simulink model "FSC_integral_KF"  (R2024b)
settings: Solver=FixedStepAuto  StartTime=0.0  StopTime=inf  FixedStep=0.001  RelTol=1e-3  EnableMultiTasking=on
undefined symbols (not defined in the file or in its folder): DiscIntNeverNeededParam, Discrete, Time
libraries: px4Sensorslib x5, px4Peripheralslib x1, ctrlSharedLib x1, cstblocks x1
settings Model: SimulationMode=external  ExtModeTrigDuration=10  Creator=ArriGE66  LastModifiedBy=xippa
settings SolverCC: PositivePriorityOrder=on
settings OptimizationCC: EnhancedBackFolding=on  PassReuseOutputArgsAs=Individual arguments  ZeroExternalMemoryAtStartup=off  ZeroInternalMemoryAtStartup=off  MaxStackSize=64  OptimizeBlockOrder=speed  DifferentSizesBufferReuse=on  OptimizationCustomize=off  EfficientTunableParamExpr=on
settings DebuggingCC: ParameterTunabilityLossMsg=error
settings HardwareCC: ProdBitPerPointer=32  ProdBitPerSizeT=32  ProdBitPerPtrDiffT=32  ProdLargestAtomicInteger=Long  ProdLargestAtomicFloat=Double  ProdWordSize=32  ProdLongLongMode=on  ProdHWDeviceType=ARM Compatible->ARM Cortex
settings SFSimCC: MATLABDynamicMemAlloc=off  SimTargetLang=C++
settings RTWCC: Description=Embedded Coder  SystemTargetFile=ert.tlc  HardwareBoard=PX4 Cube Orange  TemplateMakefile=ert_default_tmf  Toolchain=GNU Tools for PX4 Autopilots  TargetLang=C++  GPUComputeCapability=3.5
settings CodeAppCC: ForceParamTrailComments=on  IgnoreCustomStorageClasses=off  OperatorAnnotations=on  SimulinkDataObjDesc=on  SFDataObjDesc=on  InsertBlockDesc=on
settings ERTTargetCC: SupportVariableSizeSignals=on  ExtMode=on  ExtModeTransport=3  ExtModeStaticAlloc=on  ExtModeStaticAllocSize=1024  ExtModeMexFile=ext_xcp  ExtModeMexArgs=1 COM10 3000000  ExtModeIntrfLevel=Level2 - Open  InlinedParameterPlacement=Hierarchical  DynamicArrayContainerType=coder::array

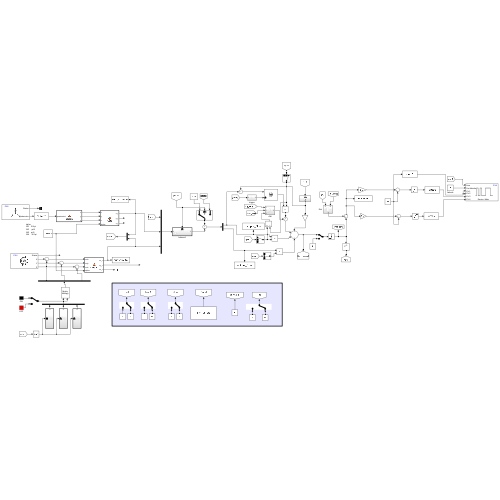
[thumbnail: Simulink's stored preview of the top-level diagram]
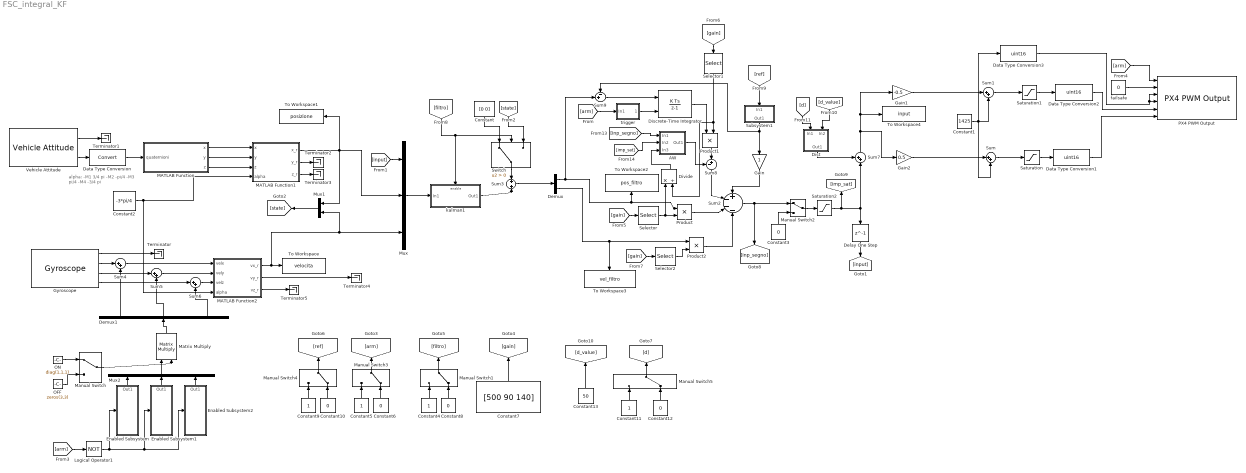
== system FSC_integral_KF ==
  note: alpha:
      | -M1    3/4 pi
      | -M2    -pi/4
      | -M3    pi/4
      | -M4    -3/4 pi
  " AW" : Subsystem
  Constant : Constant  Value=[0 0]
  Constant1 : Constant  Value=1425  SampleTime=0.01
  Constant{3,6,8,10,12} (5 alike) : Constant  Value=0
  Constant{4..5,9,11} (4 alike) : Constant
  Constant13 : Constant  Value=50
  Constant2 : Constant  Value=-3*pi/4  SampleTime=0.01
  Constant7 : Constant  Value=[500 90 140]
  Data Type Conversion : DataTypeConversion  SaturateOnIntegerOverflow=off  RndMeth=Floor
  Data Type Conversion1 : DataTypeConversion  OutDataTypeStr=uint16  SaturateOnIntegerOverflow=off  RndMeth=Floor
  Data Type Conversion2 : DataTypeConversion  OutDataTypeStr=uint16  SaturateOnIntegerOverflow=off  RndMeth=Floor
  Data Type Conversion3 : DataTypeConversion  OutDataTypeStr=uint16  SaturateOnIntegerOverflow=off  RndMeth=Floor
  Delay One Step : Delay  DelayLength=1
  Demux : Demux  Outputs=2
  Demux1 : Demux  Outputs=3
  Discrete-Time Integrator : DiscreteIntegrator  ExternalReset=level  SampleTime=-1  ICPrevOutput=DiscIntNeverNeededParam  ICPrevScaledInput=DiscIntNeverNeededParam
  Dist : Subsystem
  Divide : Product  Inputs=*/
  Enabled Subsystem : Subsystem  TreatAsAtomicUnit=on
  Enabled Subsystem1 : Subsystem  TreatAsAtomicUnit=on
  Enabled Subsystem2 : Subsystem  TreatAsAtomicUnit=on
  Gain : Gain
  Gain1 : Gain  Gain=-0.5
  Gain2 : Gain  Gain=0.5
  Gyroscope : px4Sensorslib/Gyroscope  uorbTimeStamp=off  BlockingMode=off  BlockTimeout=1e-3  sampleTime=0.01
  Logical Operator1 : Logic  Operator=NOT  AllPortsSameDT=off  OutDataTypeStr=boolean
  MATLAB Function : MATLAB Function  TreatAsAtomicUnit=on
  MATLAB Function1 : MATLAB Function  TreatAsAtomicUnit=on
  MATLAB Function2 : MATLAB Function  TreatAsAtomicUnit=on
  Manual Switch : ManualSwitch
  Manual Switch{1,3..5} (4 alike) : ManualSwitch  CurrentSetting=0
  Manual Switch2 : ManualSwitch
  Matrix Multiply : Product  Multiplication=Matrix(*)
  Mux : Mux  Inputs=3
  Mux1 : Mux  Inputs=2
  Mux2 : Mux  Inputs=3
  OFF : Constant  Value=zeros(3,3)
  ON : Constant  Value=diag(1,1,1)
  PX4 PWM Output : px4Peripheralslib/PX4 PWM Output  pwmDevice=Main  pwmChannel1_=on  pwmChannel2_=on  pwmChannel3_=on  pwmChannel4_=on  pwmChannel5_=off  pwmChannel6_=off  pwmChannel7_=off  pwmChannel8_=off
  Product : Product
  Product1 : Product
  Product2 : Product
  Saturation : Saturate  UpperLimit=1750  LowerLimit=1050
  Saturation1 : Saturate  UpperLimit=1750  LowerLimit=1050
  Saturation2 : Saturate  UpperLimit=600  LowerLimit=-600
  Selector : Selector  InputPortWidth=3  IndexOptions=Index vector (dialog)  Indices=1  OutputSizes=1
  Selector1 : Selector  InputPortWidth=3  IndexOptions=Index vector (dialog)  Indices=3  OutputSizes=1
  Selector2 : Selector  InputPortWidth=3  IndexOptions=Index vector (dialog)  Indices=2  OutputSizes=1
  Subsystem1 : Subsystem
  Sum{,1,4..6} (5 alike) : Sum  Inputs=|++
  Sum2 : Sum  Inputs=+---
  Sum3 : Sum
  Sum7 : Sum  Inputs=++|
  Sum8 : Sum  Inputs=-+|
  Sum9 : Sum  Inputs=-+|
  Switch : Switch  Criteria=u2 > Threshold  SaturateOnIntegerOverflow=off  InputSameDT=off
  Terminator{,1..5} (6 alike) : Terminator
  To Workspace : ToWorkspace  VariableName=velocita  SaveFormat=Timeseries  SampleTime=-1
  To Workspace1 : ToWorkspace  VariableName=posizione  SaveFormat=Timeseries  SampleTime=-1
  To Workspace2 : ToWorkspace  VariableName=pos_filtro  SaveFormat=Timeseries  SampleTime=-1
  To Workspace3 : ToWorkspace  VariableName=vel_filtro  SaveFormat=Timeseries  SampleTime=-1
  To Workspace4 : ToWorkspace  VariableName=input  SaveFormat=Timeseries  SampleTime=-1
  Vehicle Attitude : px4Sensorslib/Vehicle Attitude  rollRate=off  pitchRate=off  yawRate=off  quaternion=on  uorbTimeStamp=off  BlockingMode=off  BlockTimeout=0.001  sampleTime=0.01
  failsafe : Constant  Value=0  OutDataTypeStr=boolean  SampleTime=0.01
  kalman1 : Subsystem  TreatAsAtomicUnit=on
  trigger : Subsystem
  wires:
  Gain1/1 -> Sum1/1
  Data Type Conversion2/1 -> PX4 PWM Output/5
  Sum/1 -> Saturation/1
  Gain2/1 -> Sum/1
  MATLAB Function/2(y) -> MATLAB Function1/2(y)
  MATLAB Function/1(x) -> MATLAB Function1/1(x)
  MATLAB Function/3(z) -> MATLAB Function1/3(z)
  Constant1/1 -> Data Type Conversion3/1, Sum1/2, Sum/2
  Data Type Conversion1/1 -> PX4 PWM Output/6
  failsafe/1 -> PX4 PWM Output/2
  Sum1/1 -> Saturation1/1
  Vehicle Attitude/2 -> Data Type Conversion/1
  Data Type Conversion3/1 -> PX4 PWM Output/3, PX4 PWM Output/4
  MATLAB Function2/1(vx_r) -> To Workspace/1, Mux/3, Mux1/2
  Vehicle Attitude/1 -> Terminator1/1
  Saturation/1 -> Data Type Conversion1/1
  Saturation1/1 -> Data Type Conversion2/1
  MATLAB Function1/3(z_r) -> Terminator3/1
  MATLAB Function1/2(y_r) -> Terminator2/1
  MATLAB Function2/3(vz_r) -> Terminator5/1
  MATLAB Function2/2(vy_r) -> Terminator4/1
  Product/1 -> Sum2/3
  MATLAB Function1/1(x_r) -> To Workspace1/1, Mux/2, Mux1/1
  Mux/1 -> kalman1/1(In1)
  kalman1/1(Out1) -> Sum3/2
  Sum3/1 -> Demux/1
  Demux/2 -> Product2/1, To Workspace3/1
  Sum6/1 -> MATLAB Function2/3(velz)
  Gyroscope/1 -> Terminator/1
  Gyroscope/4 -> Sum6/1
  Sum4/1 -> MATLAB Function2/1(velx)
  Sum5/1 -> MATLAB Function2/2(vely)
  Constant2/1 -> MATLAB Function1/4(alpha), MATLAB Function2/4(alpha)
  Gyroscope/3 -> Sum5/1
  Gyroscope/2 -> Sum4/1
  Data Type Conversion/1 -> MATLAB Function/1(quaternioni)
  Demux1/1 -> Sum4/2
  Demux1/2 -> Sum5/2
  Demux1/3 -> Sum6/2
  Demux/1 -> Sum9/2, To Workspace2/1, Product/1
  Delay One Step/1 -> [input]
  [input] -> Mux/1
  ON/1 -> Manual Switch/1
  OFF/1 -> Manual Switch/2
  Manual Switch/1 -> Matrix Multiply/2
  Mux2/1 -> Matrix Multiply/1
  Matrix Multiply/1 -> Demux1/1
  Mux1/1 -> [state]
  Switch/1 -> Sum3/1
  [filtro] -> Switch/2, kalman1/Enable
  Constant/1 -> Switch/1
  [state] -> Switch/3
  Sum2/1 -> Manual Switch2/1, [inp_segno]
  Manual Switch2/1 -> Saturation2/1
  Constant3/1 -> Manual Switch2/2
  Enabled Subsystem/1(Out1) -> Mux2/1
  Enabled Subsystem1/1(Out1) -> Mux2/2
  Enabled Subsystem2/1(Out1) -> Mux2/3
  [arm] -> Logical Operator1/1
  Logical Operator1/1 -> Enabled Subsystem2/Enable, Enabled Subsystem1/Enable, Enabled Subsystem/Enable
  [arm] -> PX4 PWM Output/1
  Constant6/1 -> Manual Switch3/2
  Constant7/1 -> [gain]
  Manual Switch3/1 -> [arm]
  Constant5/1 -> Manual Switch3/1
  [gain] -> Selector/1
  Selector1/1 -> Divide/2, Product1/2
  Discrete-Time Integrator/1 -> Product1/1
  [gain] -> Selector1/1
  Selector2/1 -> Product2/2
  Product2/1 -> Sum2/4
  [gain] -> Selector2/1
  Constant8/1 -> Manual Switch1/2
  Manual Switch1/1 -> [filtro]
  Constant4/1 -> Manual Switch1/1
  [arm] -> trigger/1(In1)
  trigger/1(Out1) -> Discrete-Time Integrator/2
  Saturation2/1 -> [imp_sat], Sum7/2, Delay One Step/1
  Manual Switch4/1 -> [ref]
  Constant10/1 -> Manual Switch4/2
  Constant9/1 -> Manual Switch4/1
  [ref] -> Subsystem1/1(In1)
  Gain/1 -> Sum2/1
  Subsystem1/1(Out1) -> Sum9/1, Gain/1
  Dist/1(Out1) -> Sum7/1
  Constant13/1 -> [d_value]
  Constant12/1 -> Manual Switch5/2
  Constant11/1 -> Manual Switch5/1
  Manual Switch5/1 -> [d]
  [d] -> Dist/1(In1)
  [d_value] -> Dist/2(In2)
  Sum7/1 -> Gain2/1, To Workspace4/1, Gain1/1
  Product1/1 -> Sum8/2
  Sum8/1 -> Sum2/2
  [inp_segno] -> " AW"/1(In1)
  [imp_sat] -> " AW"/2(In2)
  " AW"/1(Out1) -> Sum8/1
  Selector/1 -> Product/2, Divide/1
  Divide/1 -> " AW"/3(In3)
  Sum9/1 -> Discrete-Time Integrator/1

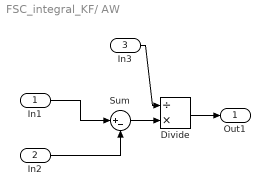
== system FSC_integral_KF/ AW ==
  In1 : Inport
  In2 : Inport  Port=2
  In3 : Inport  Port=3
  Divide : Product  Inputs=/*
  Sum : Sum  Inputs=|+-
  Out1 : Outport
  wires:
  In1/1 -> Sum/1
  In2/1 -> Sum/2
  Sum/1 -> Divide/2
  Divide/1 -> Out1/1
  In3/1 -> Divide/1

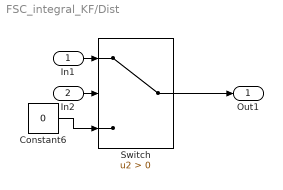
== system FSC_integral_KF/Dist ==
  In1 : Inport
  In2 : Inport  Port=2
  Constant6 : Constant  Value=0
  Switch : Switch  Criteria=u2 > Threshold  SaturateOnIntegerOverflow=off  InputSameDT=off
  Out1 : Outport
  wires:
  Constant6/1 -> Switch/3
  Switch/1 -> Out1/1
  In2/1 -> Switch/2
  In1/1 -> Switch/1

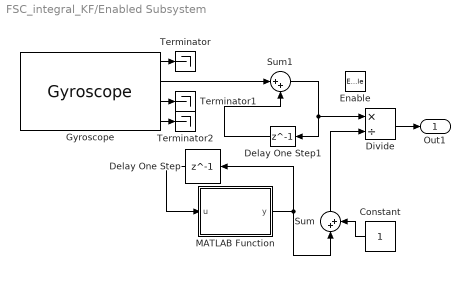
== system FSC_integral_KF/Enabled Subsystem ==
  Enable : EnablePort
  Constant : Constant
  Delay One Step : Delay  DelayLength=1
  Delay One Step1 : Delay  DelayLength=1
  Divide : Product  Inputs=*/
  Gyroscope : px4Sensorslib/Gyroscope  uorbTimeStamp=off  BlockingMode=off  BlockTimeout=1e-3  sampleTime=0.01
  MATLAB Function : MATLAB Function  TreatAsAtomicUnit=on
  Sum : Sum  Inputs=|++
  Sum1 : Sum  Inputs=|++
  Terminator : Terminator
  Terminator1 : Terminator
  Terminator2 : Terminator
  Out1 : Outport
  wires:
  Divide/1 -> Out1/1
  Sum1/1 -> Delay One Step1/1, Divide/1
  Sum/1 -> Divide/2
  Constant/1 -> Sum/2
  MATLAB Function/1(y) -> Delay One Step/1, Sum/1
  Delay One Step/1 -> MATLAB Function/1(u)
  Delay One Step1/1 -> Sum1/2
  Gyroscope/4 -> Terminator2/1
  Gyroscope/3 -> Terminator1/1
  Gyroscope/1 -> Terminator/1
  Gyroscope/2 -> Sum1/1

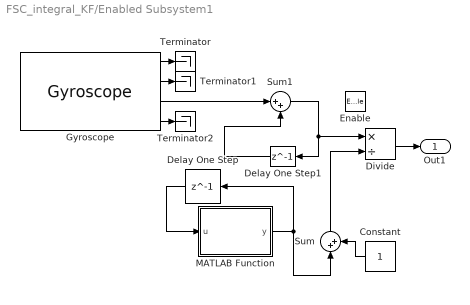
== system FSC_integral_KF/Enabled Subsystem1 ==
  Enable : EnablePort
  Constant : Constant
  Delay One Step : Delay  DelayLength=1
  Delay One Step1 : Delay  DelayLength=1
  Divide : Product  Inputs=*/
  Gyroscope : px4Sensorslib/Gyroscope  uorbTimeStamp=off  BlockingMode=off  BlockTimeout=1e-3  sampleTime=0.01
  MATLAB Function : MATLAB Function  TreatAsAtomicUnit=on
  Sum : Sum  Inputs=|++
  Sum1 : Sum  Inputs=|++
  Terminator : Terminator
  Terminator1 : Terminator
  Terminator2 : Terminator
  Out1 : Outport
  wires:
  Divide/1 -> Out1/1
  Sum1/1 -> Delay One Step1/1, Divide/1
  Sum/1 -> Divide/2
  Constant/1 -> Sum/2
  MATLAB Function/1(y) -> Delay One Step/1, Sum/1
  Delay One Step/1 -> MATLAB Function/1(u)
  Delay One Step1/1 -> Sum1/2
  Gyroscope/4 -> Terminator2/1
  Gyroscope/1 -> Terminator/1
  Gyroscope/3 -> Sum1/1
  Gyroscope/2 -> Terminator1/1

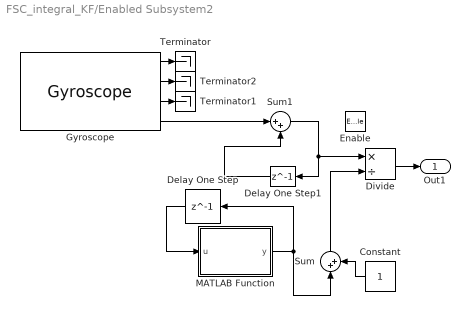
== system FSC_integral_KF/Enabled Subsystem2 ==
  Enable : EnablePort
  Constant : Constant
  Delay One Step : Delay  DelayLength=1
  Delay One Step1 : Delay  DelayLength=1
  Divide : Product  Inputs=*/
  Gyroscope : px4Sensorslib/Gyroscope  uorbTimeStamp=off  BlockingMode=off  BlockTimeout=1e-3  sampleTime=0.01
  MATLAB Function : MATLAB Function  TreatAsAtomicUnit=on
  Sum : Sum  Inputs=|++
  Sum1 : Sum  Inputs=|++
  Terminator : Terminator
  Terminator1 : Terminator
  Terminator2 : Terminator
  Out1 : Outport
  wires:
  Divide/1 -> Out1/1
  Sum1/1 -> Delay One Step1/1, Divide/1
  Sum/1 -> Divide/2
  Constant/1 -> Sum/2
  MATLAB Function/1(y) -> Delay One Step/1, Sum/1
  Delay One Step/1 -> MATLAB Function/1(u)
  Delay One Step1/1 -> Sum1/2
  Gyroscope/3 -> Terminator1/1
  Gyroscope/1 -> Terminator/1
  Gyroscope/4 -> Sum1/1
  Gyroscope/2 -> Terminator2/1

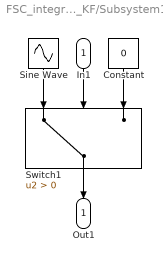
== system FSC_integral_KF/Subsystem1 ==
  In1 : Inport
  Constant : Constant  Value=0
  Sine Wave : Sin  Amplitude=0.1  SampleTime=0.01
  Switch1 : Switch  Criteria=u2 > Threshold  SaturateOnIntegerOverflow=off  InputSameDT=off
  Out1 : Outport
  wires:
  Switch1/1 -> Out1/1
  In1/1 -> Switch1/2
  Sine Wave/1 -> Switch1/1
  Constant/1 -> Switch1/3

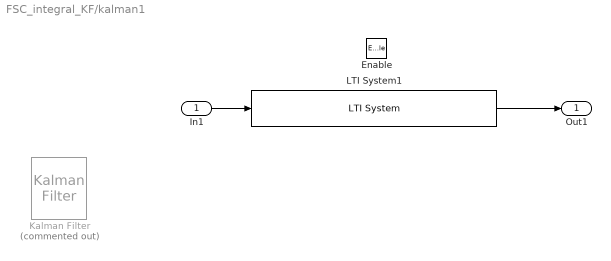
== system FSC_integral_KF/kalman1 ==
  In1 : Inport
  Enable : EnablePort
  Kalman Filter : ctrlSharedLib/Kalman Filter  Commented=on  TimeDomain=Discrete-Time  UseCurrentEstimator=on  ModelSource=LTI State-Space Variable  ModelSourceVariable=ss(0.95,1,1,0,1)  A=0.95  B=1  C=1  D=0  NumberOfStates=1  NumberOfInputs=1  NumberOfOutputs=1  InitialEstimateSource=Dialog  X0=0  P0=10  UseK=off  UseGH=off  NumberOfProcessNoiseInputs=1  G=1  TimeInvariantG=on  H=0  TimeInvariantH=on  Q=0.05  TimeInvariantQ=on  R=1  TimeInvariantR=on  N=0  TimeInvariantN=on  AddInputPort=on  AddEnablePort=off  OutputEstimatedY=off  OutputP=off  Ts=-1
  LTI System1 : cstblocks/LTI System  sys=kalmand  IC=[0 0]  PadeOrder=0
  Out1 : Outport
  wires:
  In1/1 -> LTI System1/1
  LTI System1/1 -> Out1/1

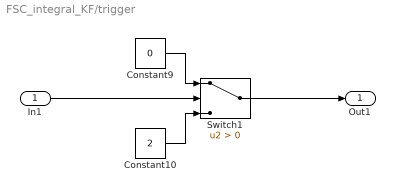
== system FSC_integral_KF/trigger ==
  In1 : Inport
  Constant10 : Constant  Value=2
  Constant9 : Constant  Value=0
  Switch1 : Switch  Criteria=u2 > Threshold  SaturateOnIntegerOverflow=off  InputSameDT=off
  Out1 : Outport
  wires:
  Constant9/1 -> Switch1/1
  Constant10/1 -> Switch1/3
  Switch1/1 -> Out1/1
  In1/1 -> Switch1/2

== matlab function FSC_integral_KF/MATLAB Function1 ==
  data: x input; y input; z input; x_r output; alpha input; y_r output; z_r output
function [x_r,y_r,z_r] = ruoto(x,y,z,alpha)
Global_POV = [x y z];
R_z = [cos(alpha), -sin(alpha), 0;
       sin(alpha), cos(alpha), 0;
       0, 0, 1];
LOCALPOV = Global_POV * R_z;
x_r = LOCALPOV(1);
y_r = LOCALPOV(2);
z_r = LOCALPOV(3);
end

== matlab function FSC_integral_KF/MATLAB Function ==
  data: x output; y output; quaternioni input; z output
function [x, y, z] = assetto(quaternioni)
    % Estrazione dei componenti del quaternione
    qw = quaternioni(1);
    qx = quaternioni(2);
    qy = quaternioni(3);
    qz = quaternioni(4);

    % Calcolo degli angoli di Eulero manualmente
    x = atan2(2*(qw*qx + qy*qz), 1 - 2*(qx^2 + qy^2)); % roll
    y = asin(2*(qw*qy - qz*qx));                          % Pitch
    z = atan2(2*(qw*qz + qx*qy), 1 - 2*(qy^2 + qz^2));   % yaw
end

== matlab function FSC_integral_KF/MATLAB Function2 ==
  data: velx input; vely input; velz input; vx_r output; alpha input; vy_r output; vz_r output
function [vx_r,vy_r,vz_r] = ruotovel(velx,vely,velz,alpha)
Global_POV = [velx vely velz];
R_z = [cos(alpha), -sin(alpha), 0;
       sin(alpha), cos(alpha), 0;
       0, 0, 1];
LOCALPOV = Global_POV * R_z;
vx_r = LOCALPOV(1);
vy_r = LOCALPOV(2);
vz_r = LOCALPOV(3);
end

== matlab function FSC_integral_KF/Enabled Subsystem/MATLAB Function ==
  data: u input; y output
function y = fcn(u)
y = u+1;

== matlab function FSC_integral_KF/Enabled Subsystem1/MATLAB Function ==
  data: u input; y output
function y = fcn(u)
y = u+1;

== matlab function FSC_integral_KF/Enabled Subsystem2/MATLAB Function ==
  data: u input; y output
function y = fcn(u)
y = u+1;
